simulink model "Motor_model_with_controller"  (R2026a)
settings: Solver=VariableStepAuto  StopTime=10
values from neighbouring files (symbols this model uses):
  D = (Kt * delta_i)/delta_omega    [MATLAB_script_data.m]
  J_new = 0.5 * 0.025 * 0.009^2 + 0.5 * robot_weight *(0.03/9.68)^2    (= 5.48357011133e-06)    [MATLAB_script_data.m]
  Kb = (delta_V - R*delta_i)/delta_omega    [MATLAB_script_data.m]
  Kp_PI = 1/G_PI_contr    [MATLAB_script_data.m]
  Kt = Kb    [MATLAB_script_data.m]
  L = tau * R    [MATLAB_script_data.m]
  R = vss_spike/iss_spike    [MATLAB_script_data.m]
  r2m = r_wheel / n    (= 0.00309917355372)    [MATLAB_script_data.m]
  tau_i = N/wc_PI    [MATLAB_script_data.m]
settings Model: Creator=sahra  LastModifiedBy=sahra

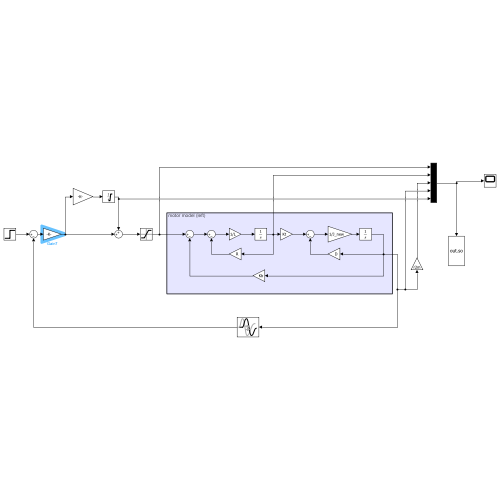
[thumbnail: Simulink's stored preview of the top-level diagram]
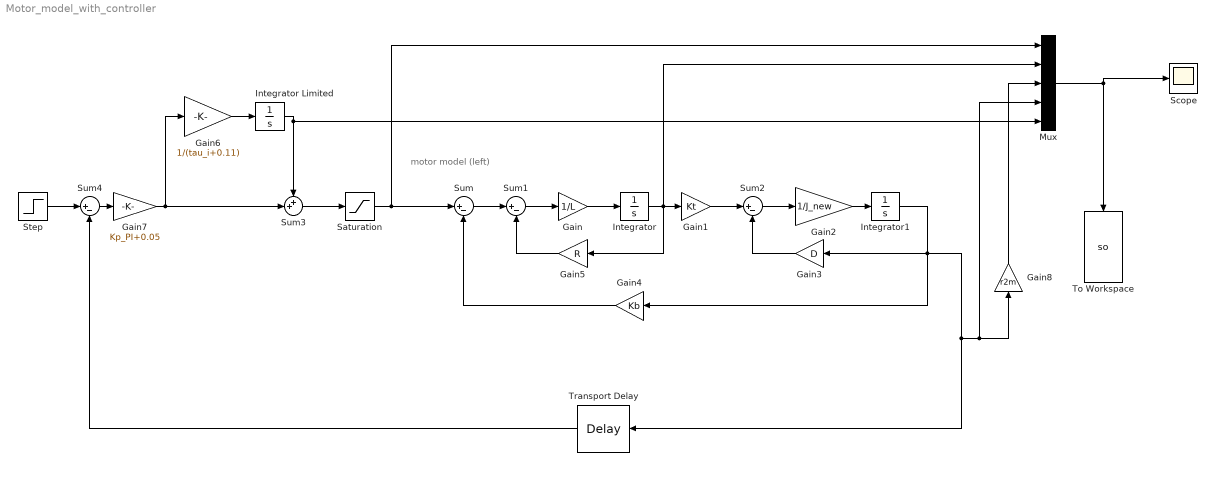
== system Motor_model_with_controller ==
  note: motor model (left)
  Gain : Gain  Gain=1/L
  Gain1 : Gain  Gain=Kt
  Gain2 : Gain  Gain=1/J_new
  Gain3 : Gain  Gain=D
  Gain4 : Gain  Gain=Kb
  Gain5 : Gain  Gain=R
  Gain6 : Gain  Gain=1/(tau_i+0.11)
  Gain7 : Gain  Gain=Kp_PI+0.05
  Gain8 : Gain  Gain=r2m
  Integrator : Integrator
  Integrator Limited : Integrator  LimitOutput=on  UpperSaturationLimit=8  LowerSaturationLimit=-8
  Integrator1 : Integrator
  Mux : Mux  Inputs=5
  Saturation : Saturate  UpperLimit=8  LowerLimit=-8
  Scope : Scope
      settings: ActiveDisplayYMinimum=-60.754208750467939  ActiveDisplayYMaximum=134.00460786451399
  Step : Step  Time=0.1  FinalValue=100  SampleTime=0
  Sum{,1..2,4} (4 alike) : Sum  Inputs=|+-
  Sum3 : Sum  Inputs=++|
  To Workspace : ToWorkspace  VariableName=so  SaveFormat=Timeseries  SampleTime=-1
  Transport Delay : TransportDelay  DelayTime=0.01
  wires:
  Sum/1 -> Sum1/1
  Sum1/1 -> Gain/1
  Gain/1 -> Integrator/1
  Integrator/1 -> Mux/2, Gain5/1, Gain1/1
  Gain1/1 -> Sum2/1
  Sum2/1 -> Gain2/1
  Gain2/1 -> Integrator1/1
  Integrator1/1 -> Gain3/1, Gain8/1, Mux/4, Transport Delay/1, Gain4/1
  Gain3/1 -> Sum2/2
  Gain4/1 -> Sum/2
  Gain5/1 -> Sum1/2
  Saturation/1 -> Mux/1, Sum/1
  Sum3/1 -> Saturation/1
  Gain6/1 -> Integrator Limited/1
  Gain7/1 -> Sum3/2, Gain6/1
  Sum4/1 -> Gain7/1
  Step/1 -> Sum4/1
  Integrator Limited/1 -> Sum3/1, Mux/5
  Mux/1 -> Scope/1, To Workspace/1
  Gain8/1 -> Mux/3
  Transport Delay/1 -> Sum4/2
